simulink model "pam_circuito_simscape"  (R2026a)
settings: Solver=ode23t  StopTime=T_sim_circ  MaxStep=max_step_circ  RelTol=1e-4
PostLoadFcn:
  | run(fullfile(fileparts(get_param(bdroot,'FileName')),'pam_simulink_init.m'))
InitFcn:
  | run(fullfile(fileparts(get_param(bdroot,'FileName')),'pam_simulink_init.m'))
values from neighbouring files (symbols this model uses):
  R1 = P.R1    [pam_simulink_init.m]
  Rgpio = P.Rgpio    [pam_simulink_init.m]
  Rprot = P.Rprot    [pam_simulink_init.m]
  Ts = P.Ts    [pam_simulink_init.m]
  usar_pwm = 0: nível médio (rápido).']))    [criar_modelos_simulink.m]
  Vmax = 3.3    [pam_simulink_init.m]
undefined symbols (not defined in the file or in its folder): R2
libraries: fl_lib x15, nesl_utility x5, simulink x1
settings Model: Creator=fonfon  LastModifiedBy=fonfon

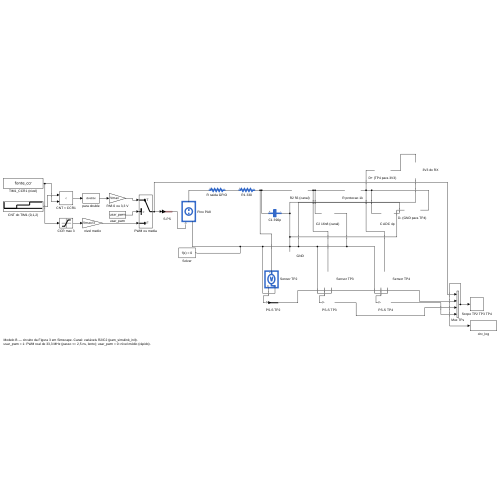
[thumbnail: Simulink's stored preview of the top-level diagram]
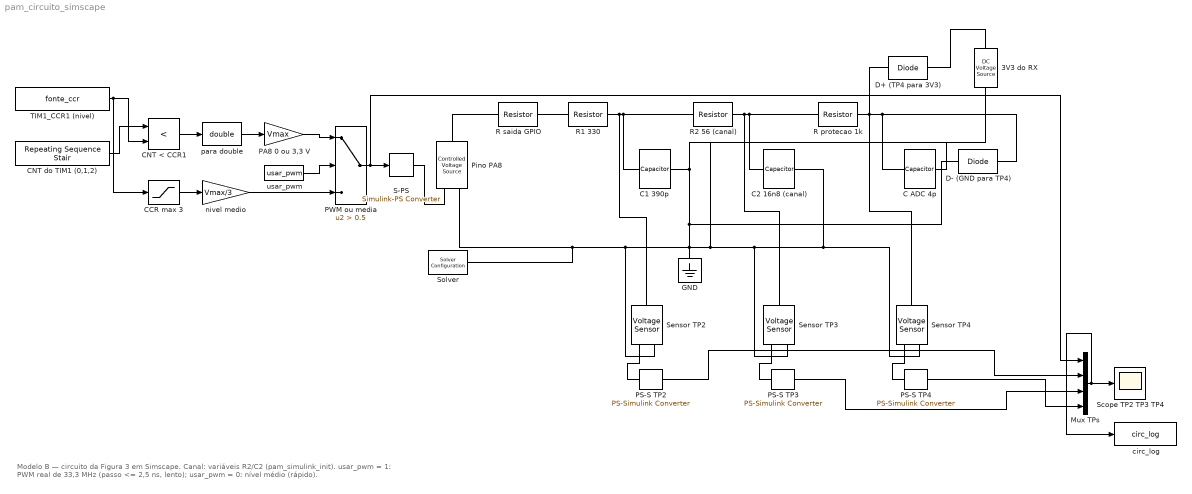
== system pam_circuito_simscape ==
  note: Modelo B — circuito da Figura 3 em Simscape. Canal: variáveis R2/C2 (pam_simulink_init).
      | usar_pwm = 1: PWM real de 33,3 MHz (passo <= 2,5 ns, lento); usar_pwm = 0: nível médio (rápido).
  3V3 do RX : fl_lib/Electrical/Electrical Sources/DC Voltage Source  v0=Vref V
  C ADC 4p : fl_lib/Electrical/Electrical Elements/Capacitor  c=C_adc F  r=1e-6 Ohm  g=0 1/Ohm  i_specify=off  i_priority=None  i=0 A  i_nominal_specify=off  i_nominal_value=1  i_nominal_unit=A  v_specify=off  v_priority=None  v=0 V  v_nominal_specify=off  v_nominal_value=1  v_nominal_unit=V  vc_specify=off  vc_priority=High  vc=0 V  vc_nominal_specify=off  vc_nominal_value=1  vc_nominal_unit=V
  C1 390p : fl_lib/Electrical/Electrical Elements/Capacitor  c=C1 F  r=1e-6 Ohm  g=0 1/Ohm  i_specify=off  i_priority=None  i=0 A  i_nominal_specify=off  i_nominal_value=1  i_nominal_unit=A  v_specify=off  v_priority=None  v=0 V  v_nominal_specify=off  v_nominal_value=1  v_nominal_unit=V  vc_specify=off  vc_priority=High  vc=0 V  vc_nominal_specify=off  vc_nominal_value=1  vc_nominal_unit=V
  C2 16n8 (canal) : fl_lib/Electrical/Electrical Elements/Capacitor  c=C2 F  r=1e-6 Ohm  g=0 1/Ohm  i_specify=off  i_priority=None  i=0 A  i_nominal_specify=off  i_nominal_value=1  i_nominal_unit=A  v_specify=off  v_priority=None  v=0 V  v_nominal_specify=off  v_nominal_value=1  v_nominal_unit=V  vc_specify=off  vc_priority=High  vc=0 V  vc_nominal_specify=off  vc_nominal_value=1  vc_nominal_unit=V
  CCR max 3 : Saturate  UpperLimit=3  LowerLimit=0
  CNT < CCR1 : RelationalOperator  Operator=<  OutDataTypeStr=boolean  RndMeth=Simplest  InputSameDT=off
  CNT do TIM1 (0,1,2) : simulink/Sources/Repeating Sequence Stair  OutValues=[0 1 2]  tsamp=10e-9  OutMin=[]  OutMax=[]  OutDataTypeStr=double  OutputDataTypeScalingMode=double  OutDataType=fixdt(0,8)  ConRadixGroup=Best Precision: Vector-wise  OutScaling=2^-12
  D+ (TP4 para 3V3) : fl_lib/Electrical/Electrical Elements/Diode  Vf=Vf_schottky V  Ron=Ron_schottky Ohm  Goff=1e-8 1/Ohm  i_specify=off  i_priority=None  i=0 A  i_nominal_specify=off  i_nominal_value=1  i_nominal_unit=A  v_specify=off  v_priority=None  v=0 V  v_nominal_specify=off  v_nominal_value=1  v_nominal_unit=V
  D- (GND para TP4) : fl_lib/Electrical/Electrical Elements/Diode  Vf=Vf_schottky V  Ron=Ron_schottky Ohm  Goff=1e-8 1/Ohm  i_specify=off  i_priority=None  i=0 A  i_nominal_specify=off  i_nominal_value=1  i_nominal_unit=A  v_specify=off  v_priority=None  v=0 V  v_nominal_specify=off  v_nominal_value=1  v_nominal_unit=V
  GND : fl_lib/Electrical/Electrical Elements/Electrical Reference
  Mux TPs : Mux
  PA8 0 ou 3,3 V : Gain  Gain=Vmax
  PS-S TP2 : nesl_utility/PS-Simulink Converter  PhysicalDomain=network_engine_domain  SubClassName=ps_output  LeftPortType=input  RightPortType=output  PseudoPeriodic=off  Frequencies=[]  VectorFormat=inherit  Unit=V  AffineConversion=off
  PS-S TP3 : nesl_utility/PS-Simulink Converter  PhysicalDomain=network_engine_domain  SubClassName=ps_output  LeftPortType=input  RightPortType=output  PseudoPeriodic=off  Frequencies=[]  VectorFormat=inherit  Unit=V  AffineConversion=off
  PS-S TP4 : nesl_utility/PS-Simulink Converter  PhysicalDomain=network_engine_domain  SubClassName=ps_output  LeftPortType=input  RightPortType=output  PseudoPeriodic=off  Frequencies=[]  VectorFormat=inherit  Unit=V  AffineConversion=off
  PWM ou media : Switch  Criteria=u2 > Threshold  Threshold=0.5  SaturateOnIntegerOverflow=off  InputSameDT=off
  Pino PA8 : fl_lib/Electrical/Electrical Sources/Controlled Voltage Source
  R protecao 1k : fl_lib/Electrical/Electrical Elements/Resistor  R=Rprot Ohm  i_specify=off  i_priority=None  i=0 A  i_nominal_specify=off  i_nominal_value=1  i_nominal_unit=A  v_specify=off  v_priority=None  v=0 V  v_nominal_specify=off  v_nominal_value=1  v_nominal_unit=V
  R saida GPIO : fl_lib/Electrical/Electrical Elements/Resistor  R=Rgpio Ohm  i_specify=off  i_priority=None  i=0 A  i_nominal_specify=off  i_nominal_value=1  i_nominal_unit=A  v_specify=off  v_priority=None  v=0 V  v_nominal_specify=off  v_nominal_value=1  v_nominal_unit=V
  R1 330 : fl_lib/Electrical/Electrical Elements/Resistor  R=R1 Ohm  i_specify=off  i_priority=None  i=0 A  i_nominal_specify=off  i_nominal_value=1  i_nominal_unit=A  v_specify=off  v_priority=None  v=0 V  v_nominal_specify=off  v_nominal_value=1  v_nominal_unit=V
  R2 56 (canal) : fl_lib/Electrical/Electrical Elements/Resistor  R=R2 Ohm  i_specify=off  i_priority=None  i=0 A  i_nominal_specify=off  i_nominal_value=1  i_nominal_unit=A  v_specify=off  v_priority=None  v=0 V  v_nominal_specify=off  v_nominal_value=1  v_nominal_unit=V
  S-PS : nesl_utility/Simulink-PS Converter  PhysicalDomain=network_engine_domain  SubClassName=ps_input  LeftPortType=input  RightPortType=output  PseudoPeriodic=off  Frequencies=[]  NoiseDistribution=none  NoiseParameters=[]  Unit=V  AffineConversion=off  FilteringAndDerivatives=provide  SimscapeFilterOrder=1  InputFilterTimeConstant=0.001  UdotUserProvided=0
  Scope TP2 TP3 TP4 : Scope
  Sensor TP2 : fl_lib/Electrical/Electrical Sensors/Voltage Sensor
  Sensor TP3 : fl_lib/Electrical/Electrical Sensors/Voltage Sensor
  Sensor TP4 : fl_lib/Electrical/Electrical Sensors/Voltage Sensor
  Solver : nesl_utility/Solver Configuration  PhysicalDomain=network_engine_domain  SubClassName=solver  LeftPortType=input  RightPortType=generic  Tones=[]  Harmonics=[]  SimulateNoise=off  Profile=off  UseLocalSampling=off  EnableSwitchedLinearOptims=on  FrequencyDomain=off  UseCCode=off  RelTol=0.001  AbsTol=0.001  MinStep=1e-09  ToWorkspace=off  RevertToSquareIcSolve=off  NumHomotopyIterations=100  PhasorMode=off  PhasorModeNumHarmonics=1  ConsistencySolver=NEWTON_XTOL_AFTER_FTOL  CanonicalOrdering=CANONICAL  OptimizeIntermediates=OPTIMIZED  IndexReductionMethod=DerivativeReplacement  DoDC=off  ResidualTolerance=1e-09  ConsistencyTolSource=GLOBAL  ConsistencyAbsTol=0.001  ConsistencyRelTol=0.001  ConsistencyTolFactor=0.001  UseLocalSolver=off  LocalSolverChoice=NE_BACKWARD_EULER_ADVANCER  ResolveIndetEquations=on  FunctionEvalNumThread=1  LocalSolverSampleTime=0.001  DoFixedCost=off  MaxNonlinIter=3  MaxModeIter=2  ComputeImpulses=off  ImpulseIterations=2  LinearAlgebra=auto  LinearAlgebraNumThread=0  EquationFormulation=NE_TIME_EF  DelaysMemoryBudget=1024  AutomaticFiltering=on  FilteringTimeConstant=0.001  PartitionStorageMethod=AS_NEEDED  PartitionMemoryBudget=1024  PartitionMethod=ROBUST  MultibodyUseLocalSolver=off  MultibodyLocalSolverChoice=ODE1  MultibodyLocalSolverSampleTime=0.001
  TIM1_CCR1 (nivel) : FromWorkspace  VariableName=fonte_ccr  SampleTime=Ts  Interpolate=off  OutputAfterFinalValue=Holding final value
  circ_log : ToWorkspace  VariableName=circ_log  SaveFormat=Structure With Time  SampleTime=5e-9
  nivel medio : Gain  Gain=Vmax/3
  para double : DataTypeConversion  OutDataTypeStr=double  SaturateOnIntegerOverflow=off  RndMeth=Floor
  usar_pwm : Constant  Value=usar_pwm
  wires:
  TIM1_CCR1 (nivel)/1 -> CNT < CCR1/2, CCR max 3/1
  CNT do TIM1 (0,1,2)/1 -> CNT < CCR1/1
  CNT < CCR1/1 -> para double/1
  para double/1 -> PA8 0 ou 3,3 V/1
  CCR max 3/1 -> nivel medio/1
  PA8 0 ou 3,3 V/1 -> PWM ou media/1
  usar_pwm/1 -> PWM ou media/2
  nivel medio/1 -> PWM ou media/3
  PWM ou media/1 -> S-PS/1, Mux TPs/1
  PS-S TP2/1 -> Mux TPs/2
  PS-S TP3/1 -> Mux TPs/3
  PS-S TP4/1 -> Mux TPs/4
  Mux TPs/1 -> Scope TP2 TP3 TP4/1, circ_log/1
  connections:
  S-PS/RConn1 -- Pino PA8/RConn1
  Pino PA8/LConn1 -- R saida GPIO/LConn1
  R saida GPIO/RConn1 -- R1 330/LConn1
  C1 390p/LConn1 -- R1 330/RConn1 -- Sensor TP2/LConn1 -- R2 56 (canal)/LConn1
  C2 16n8 (canal)/LConn1 -- R2 56 (canal)/RConn1 -- Sensor TP3/LConn1 -- R protecao 1k/LConn1
  C ADC 4p/LConn1 -- R protecao 1k/RConn1 -- D+ (TP4 para 3V3)/LConn1 -- Sensor TP4/LConn1 -- D- (GND para TP4)/RConn1
  D+ (TP4 para 3V3)/RConn1 -- 3V3 do RX/LConn1
  D- (GND para TP4)/LConn1 -- C ADC 4p/RConn1 -- C1 390p/RConn1 -- Sensor TP4/RConn2 -- C2 16n8 (canal)/RConn1 -- Sensor TP3/RConn2 -- 3V3 do RX/RConn1 -- GND/LConn1 -- Sensor TP2/RConn2 -- Solver/RConn1 -- Pino PA8/RConn2
  Sensor TP2/RConn1 -- PS-S TP2/LConn1
  Sensor TP3/RConn1 -- PS-S TP3/LConn1
  Sensor TP4/RConn1 -- PS-S TP4/LConn1
